simulink model "mppt_buck_model"  (R2023b)
settings: Solver=VariableStepAuto  StartTime=0.0  StopTime=1  RelTol=1e-3
libraries: spsSeriesRLCBranchLib x4, spsVoltageMeasurementLib x2, spsCurrentMeasurementLib x1, spsDiodeLib x1, spsMeanLib x1, spsMosfetLib x1, spsPVArrayLib x1, spsPWMGeneratorDCDCLib x1, sps_lib x1
settings Model: Creator=Suat  LastModifiedBy=Suat

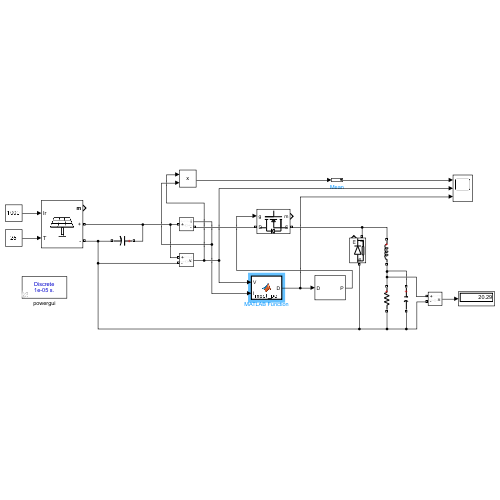
[thumbnail: Simulink's stored preview of the top-level diagram]
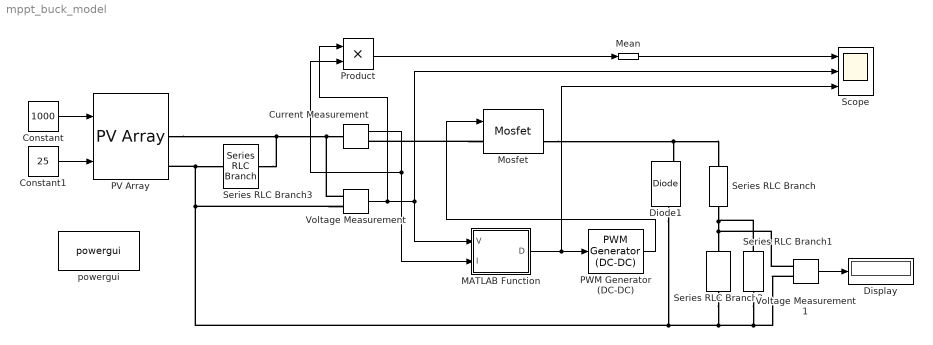
== system mppt_buck_model ==
  Constant : Constant  Value=1000
  Constant1 : Constant  Value=25
  Current Measurement : spsCurrentMeasurementLib/Current Measurement  PhasorSimulation=off  OutputType=Complex  PSBequivalent=0
  Diode1 : spsDiodeLib/Diode  Ron=0.001  Lon=0  Vf=0.8  IC=0  UseSnubber=0  Rs=500  Cs=250e-9  Measurements=on
  Display : Display
  MATLAB Function : MATLAB Function  TreatAsAtomicUnit=on
  Mean : spsMeanLib/Mean  Freq=20000  Vinit=0  Ts=1e-5
  Mosfet : spsMosfetLib/Mosfet  Ron=0.1  Lon=0  Rd=0.01  Vfd=0  IC=0  Rs=inf  Cs=0  Measurements=on
  PV Array : spsPVArrayLib/PV Array  Npar=1  Nser=1  PlotType=array @ 1000 W/m2 & specified temperatures  S_vec="[ 1000  500  100 ]"  Temp_C_vec="[ 45 25  ]"  ModuleName=User-defined  PlotWhenSelected=off  Pm=213.15  Ncell=60  Voc=36.3  Isc=7.84  Vm=29  Im=7.35  beta_Voc_pc=-0.36099  alpha_Isc_pc=0.102  beta_Voc=-0.13104  alpha_Isc=0.0079968  IL=7.8654  I0=2.9273e-10  nI=0.98119  Rsh=313.0553  Rs=0.39381  RobustModel=off  RobustCellTemperature=313.3991  BAL=on  Tc=1e-6  Tfilter=5e-5
  PWM Generator (DC-DC) : spsPWMGeneratorDCDCLib/PWM Generator (DC-DC)  Fsw=20000  Ts=1e-5
  Product : Product
  Scope : Scope  NumInputPorts=3
  Series RLC Branch : spsSeriesRLCBranchLib/Series RLC Branch  LConnTagsString=__new0  RConnTagsString=__new0  BranchType=L  Resistance=1  Inductance=1e-3  SetiL0=off  InitialCurrent=0  Capacitance=1e-6  Setx0=off  InitialVoltage=0  Measurements=None
  Series RLC Branch1 : spsSeriesRLCBranchLib/Series RLC Branch  LConnTagsString=__new0  RConnTagsString=__new0  BranchType=C  Resistance=1  Inductance=1e-3  SetiL0=off  InitialCurrent=0  Capacitance=470e-6  Setx0=off  InitialVoltage=0  Measurements=None
  Series RLC Branch2 : spsSeriesRLCBranchLib/Series RLC Branch  LConnTagsString=__new0  RConnTagsString=__new0  BranchType=R  Resistance=2  Inductance=1e-3  SetiL0=off  InitialCurrent=0  Capacitance=1e-6  Setx0=off  InitialVoltage=0  Measurements=None
  Series RLC Branch3 : spsSeriesRLCBranchLib/Series RLC Branch  LConnTagsString=__new0  RConnTagsString=__new0  BranchType=C  Resistance=1  Inductance=1e-3  SetiL0=off  InitialCurrent=0  Capacitance=4700e-6  Setx0=off  InitialVoltage=0  Measurements=None
  Voltage Measurement : spsVoltageMeasurementLib/Voltage Measurement  PhasorSimulation=off  OutputType=Complex  PSBequivalent=0
  Voltage Measurement1 : spsVoltageMeasurementLib/Voltage Measurement  PhasorSimulation=off  OutputType=Complex  PSBequivalent=0
  powergui : sps_lib/powergui  Priority=1  SimulationMode=Discrete  SampleTime=1e-5  frequency=60  Iterations=50  frequencyindice=0  Pbase=100e6  ErrMax=1e-4  UnitsV=kV  UnitsW=MW  buscounter=0  FunctionMessages=off  echomessages=off  EnableUseOfTLC=off  CurrentSourceSwitches=off  DisableSnubberDevices=off  DisableRonSwitches=off  DisableVfSwitches=off  DisplayEquations=off  AutomaticDiscreteSolvers=off  SolverType=Tustin/Backward Euler (TBE)  Interpol=off  ExternalGateDelay=off  methode=off  Ts=100  x0status=blocks  SPID=on  SwTol=0  HookPort=off  NonlinearTolerance=1e-4  nMaxIteration=100  ContinueOnMaxIteration=off  RestoreLinks=warning  ResistiveCurrentMeasurement=off  Frange=[0:2:500]  Ylog=off  Xlog=on  ShowGrid=off  save=off  variable=ZData  structure=0  ZoomFFT=off  StartTime=0.0  cycles=1  DisplayStyle=1  fundamental=60  FreqAxis=off  MaxFrequency=1000  frequencyindicesteady=1  RmsSteady=1  display=off
  wires:
  Constant/1 -> PV Array/1
  Constant1/1 -> PV Array/2
  Voltage Measurement/1 -> Product/1, MATLAB Function/1(V), Scope/2
  Current Measurement/1 -> Product/2, MATLAB Function/2(I)
  MATLAB Function/1(D) -> Scope/3, PWM Generator (DC-DC)/1
  PWM Generator (DC-DC)/1 -> Mosfet/1
  Voltage Measurement1/1 -> Display/1
  Product/1 -> Mean/1
  Mean/1 -> Scope/1
  connections:
  PV Array/RConn1 -- Series RLC Branch3/LConn1 -- Voltage Measurement/LConn1 -- Current Measurement/LConn1
  Mosfet/LConn1 -- Current Measurement/RConn1
  Voltage Measurement/LConn2 -- Voltage Measurement1/LConn2 -- Series RLC Branch1/RConn1 -- Series RLC Branch2/RConn1 -- Diode1/LConn1 -- PV Array/RConn2 -- Series RLC Branch3/RConn1
  Series RLC Branch1/LConn1 -- Series RLC Branch/RConn1 -- Voltage Measurement1/LConn1 -- Series RLC Branch2/LConn1
  Mosfet/RConn1 -- Diode1/RConn1 -- Series RLC Branch/LConn1

== matlab function mppt_buck_model/MATLAB Function ==
  data: V input; D output; I input
function D = mppt_po(V, I)
    persistent V_old P_old D_old count;
    
    if isempty(V_old)
        V_old = 36;
        P_old = 0;
        D_old = 0.5; % %50 doluluk ile başla
        count = 0;
    end
    
    % MPPT'yi her 100 simülasyon adımında bir (1 ms) güncelle
    count = count + 1;
    if count < 100
        D = D_old;
        return;
    end
    count = 0;
    
    P = V * I;
    delta_P = P - P_old;
    delta_V = V - V_old;
    
    delta_D = 0.001; % Kararlı küçük adım
    
    % Buck dönüştürücü için doğru eğim takibi:
    if delta_P > 0
        if delta_V > 0
            D = D_old - delta_D;
        else
            D = D_old + delta_D;
        end
    elseif delta_P < 0
        if delta_V > 0
            D = D_old + delta_D;
        else
            D = D_old - delta_D;
        end
    else
        D = D_old;
    end
    
    % Sınırlandırma (Geniş aralık)
    if D > 0.90
        D = 0.90;
    elseif D < 0.10
        D = 0.10;
    end
    
    V_old = V;
    P_old = P;
    D_old = D;
end
